simulink model "r2_b8a4x1kf"  (R2012b)
settings: Solver=VariableStepDiscrete  SolverMode=SingleTasking  StartTime=0.0  StopTime=1  RelTol=1e-3
undefined symbols (not defined in the file): fft_stages, n_bits_ants, n_bits_xengs
libraries: xbsIndex_r4 x22142, casper_library_misc x166, xbsReplacements_r4 x24, casper_library_delays x8, xps_library x5, casper_library_communications x4
(part 53 of 178)

== system r2_b8a4x1kf/sys3/pkt_reord_devel ==
  note: BRAM depth is
      | X int length * # antennas * # windows
  note: While reading a window out,
      | we erase the contents of that window,
      | and set the MSb (comms error).
  din : Inport
  valid_in : Inport  Port=2
  eof : Inport  Port=3
  time : Inport  Port=4
  ant : Inport  Port=5
  freq : Inport  Port=6
  flags_in : Inport  Port=7
  board_id : Inport  Port=8
  Concat : xbsIndex_r4/Concat  num_inputs=2  dbl_ovrd=off  block_type=concat
  Concat1 : xbsIndex_r4/Concat  num_inputs=2  dbl_ovrd=off  block_type=concat
  Concat2 : xbsIndex_r4/Concat  num_inputs=2  dbl_ovrd=off  block_type=concat
  Constant : xbsIndex_r4/Constant  const=0  gui_display_data_type=Fixed-point  arith_type=Unsigned  n_bits=1  bin_pt=0  preci_type=Single  exp_width=8  frac_width=24  explicit_period=on  period=1  equ=P=C  opselect=C  inp2=PCIN>>17  opr=+  inp1=P  carry=CIN  dbl_ovrd=off  block_type=constant
  Constant1 : xbsIndex_r4/Constant  const=2^ant_bits  gui_display_data_type=Fixed-point  arith_type=Unsigned  n_bits=ant_bits+1  bin_pt=0  preci_type=Single  exp_width=8  frac_width=24  explicit_period=on  period=1  equ=P=C  opselect=C  inp2=PCIN>>17  opr=+  inp1=P  carry=CIN  dbl_ovrd=off  block_type=constant
  Constant2 : xbsIndex_r4/Constant  const=1  gui_display_data_type=Fixed-point  arith_type=Unsigned  n_bits=1  bin_pt=0  preci_type=Single  exp_width=8  frac_width=24  explicit_period=on  period=1  equ=P=C  opselect=C  inp2=PCIN>>17  opr=+  inp1=P  carry=CIN  dbl_ovrd=off  block_type=constant
  Constant3 : xbsIndex_r4/Constant  const=2^(x_int_bits-n_bits_input_words)  gui_display_data_type=Fixed-point  arith_type=Unsigned  n_bits=x_int_bits  bin_pt=0  preci_type=Single  exp_width=8  frac_width=24  explicit_period=on  period=1  equ=P=C  opselect=C  inp2=PCIN>>17  opr=+  inp1=P  carry=CIN  dbl_ovrd=off  block_type=constant
  Constant4 : xbsIndex_r4/Constant  const=0  gui_display_data_type=Fixed-point  arith_type=Unsigned  n_bits=n_bits_data  bin_pt=0  preci_type=Single  exp_width=8  frac_width=24  explicit_period=on  period=1  equ=P=C  opselect=C  inp2=PCIN>>17  opr=+  inp1=P  carry=CIN  dbl_ovrd=off  block_type=constant
  Constant5 : xbsIndex_r4/Constant  const=(2^(n_bits_output_words+1))-1  gui_display_data_type=Fixed-point  arith_type=Unsigned  n_bits=2^n_bits_output_words  bin_pt=0  preci_type=Single  exp_width=8  frac_width=24  explicit_period=on  period=1  equ=P=C  opselect=C  inp2=PCIN>>17  opr=+  inp1=P  carry=CIN  dbl_ovrd=off  block_type=constant
  Delay1 : xbsIndex_r4/Delay  rst=off  infoeditControl=Selection of Reset will increase slice count due to use of real FFs and instead of SRLs  en=off  latency=3  dbl_ovrd=off  reg_retiming=on  block_type=delay
      settings: xl_area=[0, 0, 0, 0, 0, 0, 0]
  Delay{2,23..25} (4 alike) : xbsIndex_r4/Delay  rst=off  infoeditControl=Selection of Reset will increase slice count due to use of real FFs and instead of SRLs  en=off  latency=2  dbl_ovrd=off  reg_retiming=on  block_type=delay
      settings: xl_area=[0, 0, 0, 0, 0, 0, 0]
  Delay20 : xbsIndex_r4/Delay  rst=off  infoeditControl=Selection of Reset will increase slice count due to use of real FFs and instead of SRLs  en=off  latency=3  dbl_ovrd=off  reg_retiming=on  block_type=delay
      settings: xl_area=[0, 0, 0, 0, 0, 0, 0]
  Delay21 : xbsIndex_r4/Delay  rst=off  infoeditControl=Selection of Reset will increase slice count due to use of real FFs and instead of SRLs  en=off  latency=3  dbl_ovrd=off  reg_retiming=on  block_type=delay
      settings: xl_area=[0, 0, 0, 0, 0, 0, 0]
  Gateway Out{,1..8} (9 alike) : xbsIndex_r4/Gateway Out  inherit_from_input=off  hdl_port=on  timing_constraint=None  locs_specified=off  LOCs={}  UseAsDAC=off  DACChannel='1'  block_type=gatewayout
  Logical : xbsIndex_r4/Logical  logical_function=AND  inputs=2  en=off  latency=0  precision=Full  arith_type=Unsigned  n_bits=16  bin_pt=0  align_bp=on  dbl_ovrd=off  block_type=logical
  Relational : xbsIndex_r4/Relational  mode=a=b  en=off  latency=0  dbl_ovrd=off  block_type=relational
  Scope : Scope  NumInputPorts=9
      settings: YMin=-5~-5~-5~-5~-5~-5~-5~-5~-5  YMax=5~5~5~5~5~5~5~5~5
  Terminator1 : Terminator
  Terminator2 : Terminator
  ant_check : xbsIndex_r4/Assert  assert_type=on  type_source=Explicitly  gui_display_data_type=Fixed-point  arith_type=Unsigned  n_bits=ant_bits  bin_pt=0  preci_type=Single  exp_width=8  frac_width=24  assert_rate=off  rate_source=Explicitly  period=1  output_port=on  block_type=assert
  bus_expand : Subsystem  AncestorBlock=casper_library_flow_control/bus_expand  mask(bus_expand){mode=divisions of arbitrary size, outputNum=1, outputWidth=[2^n_bits_output_words, (2^n_bits_output_words)*n_bits_data], outputBinaryPt=[0, 0], outputArithmeticType=[0, 0], show_format=off, outputToWorkspace=off, variablePrefix=out, outputToModelAsWell=on}
      mask prompts: outputNum "Number of outputs:"; outputWidth "Output width [msb ... lsb]:"; outputBinaryPt "Output binary point position [msb ... lsb]:"; outputArithmeticType "Output arithmetic type (ufix=0, fix=1, bool=2) [msb ... lsb]:"; show_format "Print format string?"; outputToWorkspace "Output to workspace?"; variablePrefix "Variable name prefix:"; outputToModelAsWell "Output to model as well?"
      mask help:
      | Expands a 'bus' made using a bus_create or Xilinx
      | concat block.
      | The input will be divided into the specified number
      | of outputs with the specified arithmetic types.
      | Divisions are made from most significant bit.
      mask init: same as r2_b8a4x1kf/bus_expand
      settings: AttributesFormatString=2 outputs
      mask TypeOptions mode: divisions of equal size | divisions of arbitrary size
      mask Callback mode: bus_expand_callback();
      mask Callback outputWidth: bus_expand_callback();
      mask Callback outputToWorkspace: bus_expand_callback();
  bus_replicate : Subsystem  AncestorBlock=casper_library_bus/bus_replicate  mask(bus_replicate){replication=2^n_bits_output_words, latency=0, misc=off, implementation=behavioral}
      mask prompts: replication "replication factor"; misc "misc support"; implementation "delay implementation"
      mask help: Output bus formed by replicating input bus a number of times
      mask init:
      | bus_replicate_init(gcb, ...
      |     'replication', replication, ...
      |     'latency', latency, ...
      |     'implementation', implementation, ...
      |     'misc', misc);
      mask TypeOptions implementation: core | behavioral
  data_buffer : xbsIndex_r4/Dual Port RAM  depth=2^x_int_bits * 2^ant_bits * 2^window_bits  initVector=0  distributed_mem=Block RAM  init_a=0  init_b=0  rst_a=off  rst_b=off  en_a=off  en_b=off  latency=3  write_mode_A=Read Before Write  write_mode_B=Read Before Write  dbl_ovrd=off  optimize=Area  block_type=dpram
      settings: xl_area=[0, 0, 0, 0, 0, 0, 0]  block_version=10.1.3
  data_check : xbsIndex_r4/Assert  assert_type=on  type_source=Explicitly  gui_display_data_type=Fixed-point  arith_type=Unsigned  n_bits=n_bits_data * 2^n_bits_input_words  bin_pt=0  preci_type=Single  exp_width=8  frac_width=24  assert_rate=off  rate_source=Explicitly  period=1  output_port=on  block_type=assert
  flag_buffer : xbsIndex_r4/Dual Port RAM  depth=2^ant_bits * 2^window_bits  initVector=zeros(1, 2^ant_bits * 2^window_bits)  distributed_mem=Distributed memory  init_a=0  init_b=0  rst_a=off  rst_b=off  en_a=off  en_b=off  latency=3  write_mode_A=Read After Write  write_mode_B=Read After Write  dbl_ovrd=off  optimize=Area  block_type=dpram
  flag_check : xbsIndex_r4/Assert  assert_type=on  type_source=Explicitly  gui_display_data_type=Fixed-point  arith_type=Unsigned  n_bits=n_bits_flag  bin_pt=0  preci_type=Single  exp_width=8  frac_width=24  assert_rate=off  rate_source=Explicitly  period=1  output_port=on  block_type=assert
  freq_check : xbsIndex_r4/Assert  assert_type=on  type_source=Explicitly  gui_display_data_type=Fixed-point  arith_type=Unsigned  n_bits=chan_bits-xeng_bits  bin_pt=0  preci_type=Single  exp_width=8  frac_width=24  assert_rate=off  rate_source=Explicitly  period=1  output_port=on  block_type=assert
  input_control : Subsystem
  msbs0 : xbsIndex_r4/Slice  nbits=window_bits + ant_bits  boolean_output=off  mode=Upper Bit Location + Width  bit1=0  base1=MSB of Input  bit0=0  base0=LSB of Input  dbl_ovrd=off  block_type=slice
  msbs1 : xbsIndex_r4/Slice  nbits=window_bits+ant_bits  boolean_output=off  mode=Upper Bit Location + Width  bit1=0  base1=MSB of Input  bit0=0  base0=LSB of Input  dbl_ovrd=off  block_type=slice
  munge : Subsystem  AncestorBlock=casper_library_flow_control/munge  mask(munge){divisions=1 + 2^n_bits_input_words, div_size=[1, repmat(n_bits_data, 1, 2^n_bits_input_words)], order=reshape([zeros(1, 2^n_bits_input_words); 1:2^n_bits_input_words], 1, 2^(n_bits_input_words+1)), arith_type_out=Unsigned, bin_pt_out=0}
      mask prompts: divisions "Number of divisions"; div_size "Division size (bits)"; order "Division packing order"; arith_type_out "Output arithmetic type"; bin_pt_out "Output binary point"
      mask help: Splits an input bus into the specified number of divisions and then recombines them in the order specified (most significant division = 0,least = number divisions-1)
      mask init:
      | munge_init(gcb, ...
      |     'divisions', divisions, ...
      |     'div_size', div_size, ...
      |     'order', order, ...
      |     'arith_type_out', arith_type_out, ...
      |     'bin_pt_out', bin_pt_out);
      settings: AttributesFormatString=|
      | split:[1 32 32]
      | join:[0 1 0 2]
      | Unsigned [66,0]
      mask TypeOptions arith_type_out: Unsigned | Signed  (2's comp) | Floating-point
  munge1 : Subsystem  AncestorBlock=casper_library_flow_control/munge  mask(munge){divisions=2^(n_bits_output_words+1), div_size=reshape([ones(1, 2^n_bits_output_words); repmat(n_bits_data, 1 ,2^n_bits_output_words)], 1, 2^(n_bits_output_words+1)), order=[[0:2:2^(n_bits_output_words+1)-2], [1:2:2^(n_bits_output_words+1)-1]], arith_type_out=Unsigned, bin_pt_out=0}
      mask prompts: divisions "Number of divisions"; div_size "Division size (bits)"; order "Division packing order"; arith_type_out "Output arithmetic type"; bin_pt_out "Output binary point"
      mask help: Splits an input bus into the specified number of divisions and then recombines them in the order specified (most significant division = 0,least = number divisions-1)
      mask init:
      | munge_init(gcb, ...
      |     'divisions', divisions, ...
      |     'div_size', div_size, ...
      |     'order', order, ...
      |     'arith_type_out', arith_type_out, ...
      |     'bin_pt_out', bin_pt_out);
      settings: AttributesFormatString=|
      | split:[1 32]
      | join:[0 1]
      | Unsigned [33,0]
      mask TypeOptions arith_type_out: Unsigned | Signed  (2's comp) | Floating-point
  output_control : Subsystem
  time_check : xbsIndex_r4/Assert  assert_type=on  type_source=Explicitly  gui_display_data_type=Fixed-point  arith_type=Unsigned  n_bits=n_bits_timestamp  bin_pt=0  preci_type=Single  exp_width=8  frac_width=24  assert_rate=off  rate_source=Explicitly  period=1  output_port=on  block_type=assert
  time_freq_unpack : Subsystem
  sync_out : Outport
  data_out : Outport  Port=2
  valid_out : Outport  Port=3
  time_out : Outport  Port=4
  freq_out : Outport  Port=5
  flags_out : Outport  Port=6
  recvd : Outport  Port=7
  packet_discarded : Outport  Port=8
  mcnt_timeout : Outport  Port=9
  wires:
  ant_check/1 -> input_control/6(src)
  eof/1 -> input_control/4(eof)
  valid_in/1 -> input_control/3(valid)
  flag_check/1 -> input_control/2(flag_in)
  data_check/1 -> input_control/1(data_in)
  input_control/7(mcnt_timeout) -> mcnt_timeout/1
  flag_buffer/2 -> flags_out/1, Gateway Out8/1
  flag_buffer/1 -> Terminator2/1
  Delay24/1 -> Gateway Out2/1, data_buffer/4, msbs0/1
  Gateway Out8/1 -> Scope/9
  Gateway Out5/1 -> Scope/6
  Gateway Out2/1 -> Scope/3
  Gateway Out3/1 -> Scope/4
  Gateway Out6/1 -> Scope/7
  Gateway Out/1 -> Scope/1
  Gateway Out1/1 -> Scope/2
  Gateway Out7/1 -> Scope/8
  Gateway Out4/1 -> Scope/5
  Logical/1 -> recvd/1
  Relational/1 -> Logical/2
  freq_check/1 -> Concat2/2
  time_check/1 -> Concat2/1
  Constant5/1 -> Relational/1
  bus_expand/1(msb_out2) -> Relational/2
  bus_expand/2(lsb_out1) -> data_out/1
  munge1/1(dout) -> bus_expand/1(bus_in)
  time/1 -> time_check/1
  Concat1/1 -> bus_replicate/1(in)
  bus_replicate/1(out) -> data_buffer/2
  Constant/1 -> Concat1/1
  Constant4/1 -> Concat1/2
  munge/1(dout) -> data_buffer/5
  input_control/6(discarding) -> packet_discarded/1
  Delay23/1 -> Concat/2
  Concat/1 -> munge/1(din)
  Constant2/1 -> Concat/1
  msbs1/1 -> flag_buffer/4, Gateway Out6/1
  Delay2/1 -> flag_buffer/2, Gateway Out7/1
  input_control/5(wr_flag) -> Delay2/1
  msbs0/1 -> flag_buffer/1, Gateway Out4/1
  Concat2/1 -> input_control/5(time_freq)
  flags_in/1 -> flag_check/1
  ant/1 -> ant_check/1
  din/1 -> data_check/1
  board_id/1 -> time_freq_unpack/2(xeng_id)
  input_control/4(we) -> Delay25/1
  input_control/2(wr_addr) -> Delay24/1
  output_control/2(rd_en) -> data_buffer/3, Gateway Out1/1, Delay21/1
  output_control/3(rd_addr) -> Gateway Out/1, data_buffer/1, msbs1/1
  Delay21/1 -> valid_out/1, Logical/1
  Delay20/1 -> sync_out/1
  data_buffer/2 -> Terminator1/1
  data_buffer/1 -> munge1/1(din)
  output_control/1(gen_sync) -> Delay20/1
  input_control/3(wr_data) -> Delay23/1
  input_control/1(maxcnt) -> output_control/1(maxcnt)
  Delay25/1 -> data_buffer/6, Gateway Out3/1, flag_buffer/3, Gateway Out5/1
  output_control/4(rd_timefreq) -> Delay1/1
  Constant3/1 -> input_control/7(pkt_size)
  Constant1/1 -> input_control/8(n_src)
  freq/1 -> freq_check/1
  time_freq_unpack/1(time) -> time_out/1
  Delay1/1 -> time_freq_unpack/1(din)
  time_freq_unpack/2(freq) -> freq_out/1

== system r2_b8a4x1kf/sys3/pre_process ==
  note: slice off the bits of timestamp
      | that matter
  note: check that the
      | frequency has gone
      | to the correct ip
  note: HDRs are:
      | 1. Timestamp,
      | 2. feng_id,
      | 3. feng_satus,
      | 4. frequency
  note: application 32-47
      | reserved 24-31
      | fengine 8-23
      | digitiser 0-7
  data_in : Inport
  valid_in : Inport  Port=2
  eof_in : Inport  Port=3
  spead_err : Inport  Port=4
  spead_time48 : Inport  Port=5
  spead_fengid : Inport  Port=6
  spead_flags : Inport  Port=7
  heap_offset : Inport  Port=8
  xeng_id : Inport  Port=9
  freq_offset : Inport  Port=10
  Concat : xbsIndex_r4/Concat  num_inputs=15  dbl_ovrd=off  block_type=concat
  Concat1 : xbsIndex_r4/Concat  num_inputs=6  dbl_ovrd=off  block_type=concat
  Constant : xbsIndex_r4/Constant  const=0  gui_display_data_type=Boolean  arith_type=Boolean  n_bits=1  bin_pt=0  preci_type=Single  exp_width=8  frac_width=24  explicit_period=on  period=1  equ=P=C  opselect=C  inp2=PCIN>>17  opr=+  inp1=P  carry=CIN  dbl_ovrd=off  block_type=constant
  Delay{1..10} (10 alike) : xbsIndex_r4/Delay  rst=off  infoeditControl=Selection of Reset will increase slice count due to use of real FFs and instead of SRLs  en=off  latency=1  dbl_ovrd=off  reg_retiming=on  block_type=delay
      settings: xl_area=[0, 0, 0, 0, 0, 0, 0]
  Delay13 : xbsIndex_r4/Delay  rst=off  infoeditControl=Selection of Reset will increase slice count due to use of real FFs and instead of SRLs  en=on  latency=1  dbl_ovrd=off  reg_retiming=on  block_type=delay
      settings: xl_area=[0, 0, 0, 0, 0, 0, 0]
  Gateway Out{1,8,10..13} (6 alike) : xbsIndex_r4/Gateway Out  inherit_from_input=off  hdl_port=off  timing_constraint=None  locs_specified=off  LOCs={}  UseAsDAC=off  DACChannel='1'  block_type=gatewayout
      settings: infoedit="Gateway out block.  Converts Xilinx fixed point inputs into ouputs of type Simulink integer, double, or fixed point.<P><P>Hardware notes:  In hardware these blocks become top level output ports or are discarded, depending on how they are configured."  xl_area=[0, 0, 0, 0, 0, 0, 0]  block_version=10.1.3
  Inverter : xbsIndex_r4/Inverter  en=off  latency=0  dbl_ovrd=off  block_type=inv
      settings: block_version=11.4
  Logical : xbsIndex_r4/Logical  logical_function=OR  inputs=7  en=off  latency=0  precision=Full  arith_type=Unsigned  n_bits=16  bin_pt=0  align_bp=on  dbl_ovrd=off  block_type=logical
  Logical1 : xbsIndex_r4/Logical  logical_function=AND  inputs=2  en=off  latency=0  precision=Full  arith_type=Unsigned  n_bits=8  bin_pt=2  align_bp=on  dbl_ovrd=off  block_type=logical
      settings: xl_area=[0, 0, 0, 0, 0, 0, 0]
  Logical{2,4..6} (4 alike) : xbsIndex_r4/Logical  logical_function=OR  inputs=2  en=off  latency=0  precision=Full  arith_type=Unsigned  n_bits=16  bin_pt=0  align_bp=on  dbl_ovrd=off  block_type=logical
  Logical3 : xbsIndex_r4/Logical  logical_function=AND  inputs=2  en=off  latency=0  precision=Full  arith_type=Unsigned  n_bits=8  bin_pt=2  align_bp=on  dbl_ovrd=off  block_type=logical
      settings: xl_area=[0, 0, 0, 0, 0, 0, 0]
  Slice : xbsIndex_r4/Slice  nbits=1  boolean_output=off  mode=Two Bit Locations  bit1=0  base1=MSB of Input  bit0=(freq_bits+1) + acc_bits  base0=LSB of Input  dbl_ovrd=off  block_type=slice
  Slice{1,4..7} (5 alike) : xbsIndex_r4/Slice  nbits=1  boolean_output=on  mode=Lower Bit Location + Width  bit1=0  base1=MSB of Input  bit0=0  base0=LSB of Input  dbl_ovrd=off  block_type=slice
  Slice9 : xbsIndex_r4/Slice  nbits=ant_bits  boolean_output=off  mode=Lower Bit Location + Width  bit1=0  base1=MSB of Input  bit0=0  base0=LSB of Input  dbl_ovrd=off  block_type=slice
      settings: block_version=10.1.3
  Terminator{,1..3} (4 alike) : Terminator
  bus_expand : Subsystem  AncestorBlock=casper_library_flow_control/bus_expand  mask(bus_expand){mode=divisions of arbitrary size, outputNum=1, outputWidth=[16 8 16 8], outputBinaryPt=0, outputArithmeticType=0, show_format=off, outputToWorkspace=off, variablePrefix=out, outputToModelAsWell=on}
      mask prompts: outputNum "Number of outputs:"; outputWidth "Output width [msb ... lsb]:"; outputBinaryPt "Output binary point position [msb ... lsb]:"; outputArithmeticType "Output arithmetic type (ufix=0, fix=1, bool=2) [msb ... lsb]:"; show_format "Print format string?"; outputToWorkspace "Output to workspace?"; variablePrefix "Variable name prefix:"; outputToModelAsWell "Output to model as well?"
      mask help:
      | Expands a 'bus' made using a bus_create or Xilinx
      | concat block.
      | The input will be divided into the specified number
      | of outputs with the specified arithmetic types.
      | Divisions are made from most significant bit.
      mask init: same as r2_b8a4x1kf/bus_expand
      settings: AttributesFormatString=4 outputs
      mask TypeOptions mode: divisions of equal size | divisions of arbitrary size
      mask Callback mode: bus_expand_callback();
      mask Callback outputWidth: bus_expand_callback();
      mask Callback outputToWorkspace: bus_expand_callback();
  bus_expand1 : Subsystem  AncestorBlock=casper_library_flow_control/bus_expand  mask(bus_expand){mode=divisions of arbitrary size, outputNum=1, outputWidth=[4 1 1 1 1], outputBinaryPt=[0 0 0 0 0], outputArithmeticType=[0 0 0 0 0], show_format=off, outputToWorkspace=off, variablePrefix=out, outputToModelAsWell=on}
      mask prompts: outputNum "Number of outputs:"; outputWidth "Output width [msb ... lsb]:"; outputBinaryPt "Output binary point position [msb ... lsb]:"; outputArithmeticType "Output arithmetic type (ufix=0, fix=1, bool=2) [msb ... lsb]:"; show_format "Print format string?"; outputToWorkspace "Output to workspace?"; variablePrefix "Variable name prefix:"; outputToModelAsWell "Output to model as well?"
      mask help:
      | Expands a 'bus' made using a bus_create or Xilinx
      | concat block.
      | The input will be divided into the specified number
      | of outputs with the specified arithmetic types.
      | Divisions are made from most significant bit.
      mask init: same as r2_b8a4x1kf/bus_expand
      settings: AttributesFormatString=5 outputs
      mask TypeOptions mode: divisions of equal size | divisions of arbitrary size
      mask Callback mode: bus_expand_callback();
      mask Callback outputWidth: bus_expand_callback();
      mask Callback outputToWorkspace: bus_expand_callback();
  bus_expand2 : Subsystem  AncestorBlock=casper_library_flow_control/bus_expand  mask(bus_expand){mode=divisions of arbitrary size, outputNum=1, outputWidth=[5 1 1 1 1 1 1 1 1 1 1 1], outputBinaryPt=[0 0 0 0 0 0 0 0 0 0 0 0], outputArithmeticType=[0 0 0 0 0 0 0 0 0 0 0 0], show_format=off, outputToWorkspace=off, variablePrefix=out, outputToModelAsWell=on}
      mask prompts: outputNum "Number of outputs:"; outputWidth "Output width [msb ... lsb]:"; outputBinaryPt "Output binary point position [msb ... lsb]:"; outputArithmeticType "Output arithmetic type (ufix=0, fix=1, bool=2) [msb ... lsb]:"; show_format "Print format string?"; outputToWorkspace "Output to workspace?"; variablePrefix "Variable name prefix:"; outputToModelAsWell "Output to model as well?"
      mask help:
      | Expands a 'bus' made using a bus_create or Xilinx
      | concat block.
      | The input will be divided into the specified number
      | of outputs with the specified arithmetic types.
      | Divisions are made from most significant bit.
      mask init: same as r2_b8a4x1kf/bus_expand
      settings: AttributesFormatString=12 outputs
      mask TypeOptions mode: divisions of equal size | divisions of arbitrary size
      mask Callback mode: bus_expand_callback();
      mask Callback outputWidth: bus_expand_callback();
      mask Callback outputToWorkspace: bus_expand_callback();
  correct_ip : xbsIndex_r4/Relational  mode=a=b  en=off  latency=1  dbl_ovrd=off  block_type=relational
      settings: xl_area=[0, 0, 0, 0, 0, 0, 0]  block_version=10.1.3
  correct_xengine : xbsIndex_r4/Relational  mode=a=b  en=off  latency=1  dbl_ovrd=off  block_type=relational
      settings: xl_area=[0, 0, 0, 0, 0, 0, 0]  block_version=10.1.3
  dest_ip : xbsIndex_r4/Slice  nbits=xeng_bits-share_bits  boolean_output=off  mode=Upper Bit Location + Width  bit1=0  base1=MSB of Input  bit0=freq_bits-xeng_bits  base0=LSB of Input  dbl_ovrd=off  block_type=slice
      settings: block_version=10.1.3
  edge_detect : casper_library_misc/edge_detect  edge=Rising  polarity=Active High  x_in=[0 0.08 0.08 0.16 0.16 0.24 0.24 0.32 0.32 0.4]  y_in="[-1 -1  1  1  1  1  1  1  1  1]"  x_out=[0.6 0.68 0.68 0.76 0.76 0.84 0.84 0.92 0.92 1]  y_out="[-1 -1  1  1 -1 -1 -1 -1 -1 -1]"
  freq : xbsIndex_r4/Slice  nbits=freq_bits - xeng_bits  boolean_output=off  mode=Lower Bit Location + Width  bit1=0  base1=LSB of Input  bit0=acc_bits - 1 + 3  base0=LSB of Input  dbl_ovrd=off  block_type=slice
      settings: block_version=10.1.3
  freq_id : xbsIndex_r4/Slice  nbits=xeng_bits  boolean_output=off  mode=Lower Bit Location + Width  bit1=freq_bits  base1=LSB of Input  bit0=freq_bits-xeng_bits  base0=LSB of Input  dbl_ovrd=off  block_type=slice
      settings: block_version=10.1.3
  pre_proc : Scope  NumInputPorts=6
      settings: TimeRange=1  YMin=1.06962e+15~0~142.5~3.8~-1~0  YMax=1.18222e+15~1~157.5~4.2~1~1  SaveName=ScopeData10
  x_ip : xbsIndex_r4/Slice  nbits=xeng_bits-share_bits  boolean_output=off  mode=Upper Bit Location + Width  bit1=0  base1=MSB of Input  bit0=freq_bits-xeng_bits  base0=LSB of Input  dbl_ovrd=off  block_type=slice
      settings: block_version=10.1.3
  xeng : xbsIndex_r4/Slice  nbits=xeng_bits  boolean_output=off  mode=Lower Bit Location + Width  bit1=0  base1=MSB of Input  bit0=0  base0=LSB of Input  dbl_ovrd=off  block_type=slice
      settings: block_version=10.1.3
  data_out : Outport
  valid : Outport  Port=2
  eof_out : Outport  Port=3
  timestamp : Outport  Port=4
  feng_id : Outport  Port=5
  freq_out : Outport  Port=6
  spead_err_out : Outport  Port=7
  ip_dest_err : Outport  Port=8
  flags_out : Outport  Port=9
  err_bundle : Outport  Port=10
  wires:
  Gateway Out1/1 -> pre_proc/6
  Delay6/1 -> Gateway Out13/1
  Delay3/1 -> Logical3/1, Gateway Out10/1, Logical1/1
  Gateway Out10/1 -> pre_proc/2
  Gateway Out11/1 -> pre_proc/1
  Gateway Out12/1 -> pre_proc/3
  Gateway Out13/1 -> pre_proc/4
  Gateway Out8/1 -> pre_proc/5
  Logical1/1 -> edge_detect/1
  Inverter/1 -> Logical1/2
  xeng_id/1 -> xeng/1
  heap_offset/1 -> freq/1
  Logical3/1 -> valid/1, Gateway Out8/1
  valid_in/1 -> Delay3/1, Delay13/2
  xeng/1 -> Delay1/1, correct_xengine/2, x_ip/1
  freq_id/1 -> correct_xengine/1, Delay6/1, dest_ip/1
  Delay1/1 -> Gateway Out11/1
  Delay2/1 -> Gateway Out12/1
  eof_in/1 -> Delay7/1
  data_in/1 -> Delay5/1
  Delay5/1 -> data_out/1
  spead_fengid/1 -> Slice9/1
  Delay4/1 -> freq_out/1
  Delay7/1 -> eof_out/1
  Delay8/1 -> spead_err_out/1
  Delay9/1 -> timestamp/1
  Delay10/1 -> feng_id/1
  spead_err/1 -> Delay8/1
  spead_time48/1 -> Slice/1
  Slice/1 -> Delay9/1
  freq/1 -> Delay4/1, Delay2/1
  Slice9/1 -> Delay10/1
  spead_flags/1 -> Delay13/1
  Delay13/1 -> bus_expand/1(bus_in)
  bus_expand/4(lsb_out1) -> bus_expand1/1(bus_in)
  bus_expand/3(out2) -> bus_expand2/1(bus_in)
  bus_expand/2(out3) -> Terminator/1
  bus_expand/1(msb_out4) -> Terminator1/1
  bus_expand1/1(msb_out5) -> Terminator2/1
  bus_expand2/1(msb_out12) -> Terminator3/1
  bus_expand2/6(out7) -> Concat/5, Logical/1
  bus_expand2/7(out6) -> Logical/2, Concat/6
  bus_expand2/8(out5) -> Concat/7, Logical/3
  bus_expand2/9(out4) -> Concat/8, Logical/4
  bus_expand2/10(out3) -> Logical/5, Concat/9
  bus_expand2/11(out2) -> Logical/6, Concat/10
  bus_expand2/12(lsb_out1) -> Logical/7, Concat/11
  Concat/1 -> flags_out/1
  Logical/1 -> Slice5/1
  Constant/1 -> [pre_feng_chk_err]
  bus_expand2/2(out11) -> Logical2/1, Concat/1
  bus_expand2/3(out10) -> Logical2/2, Concat/2
  bus_expand2/4(out9) -> Concat/3, Logical4/1
  bus_expand2/5(out8) -> Logical4/2, Concat/4
  Logical4/1 -> Slice4/1
  Logical2/1 -> Slice1/1
  bus_expand1/2(out4) -> Concat/12, Logical5/1
  bus_expand1/3(out3) -> Concat/13, Logical5/2
  Logical6/1 -> Slice7/1
  bus_expand1/4(out2) -> Logical6/1, Concat/14
  bus_expand1/5(lsb_out1) -> Concat/15, Logical6/2
  Logical5/1 -> Slice6/1
  Slice1/1 -> [pre_feng_qdr_err]
  Slice4/1 -> [pre_fft_err]
  Slice5/1 -> [pre_feng_rx_err]
  Slice6/1 -> [pre_adc_err]
  Slice7/1 -> [pre_ndiode_en]
  correct_xengine/1 -> Logical3/2
  edge_detect/1 -> Gateway Out1/1, ip_dest_err/1
  dest_ip/1 -> correct_ip/1
  x_ip/1 -> correct_ip/2
  correct_ip/1 -> Inverter/1
  Concat1/1 -> err_bundle/1
  [pre_adc_err] -> Concat1/5
  [pre_feng_rx_err] -> Concat1/4
  [pre_fft_err] -> Concat1/3
  [pre_feng_chk_err] -> Concat1/1
  [pre_ndiode_en] -> Concat1/6
  [pre_feng_qdr_err] -> Concat1/2
  freq_offset/1 -> freq_id/1
